simulink model "Test_Estimation_Effects"  (R2026a)
settings: Solver=FixedStepAuto  StopTime=SIM.StopTime  FixedStep=SIM.FixedStepSize
undefined symbols (not defined in the file): AP, AP_SRC, CMD, DES, DiscIntNeverNeededParam, drawAircraft, EST, F, Light, LIM, MAV, MIL, plotter, SIM, TRIM, WIND
libraries: simulink x11, matrix_library x2, aerolibwind2 x1
(part 1 of 2)
settings Model: Creator=emrec  LastModifiedBy=emrec

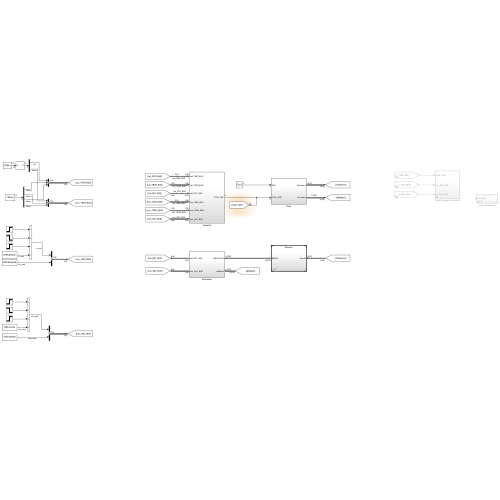
[thumbnail: Simulink's stored preview of the top-level diagram]
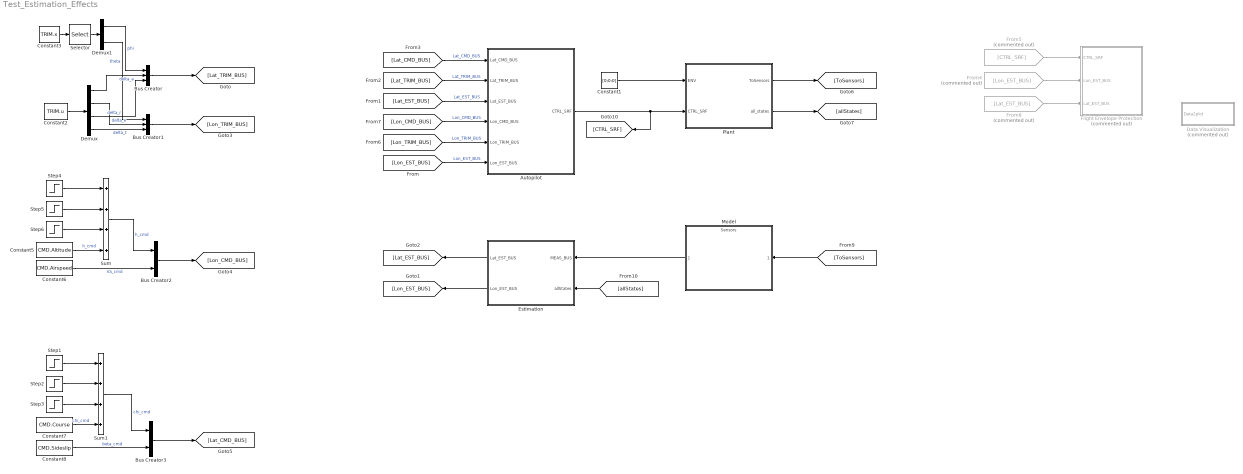
== system Test_Estimation_Effects ==
  Autopilot : Subsystem
  Bus Creator : BusCreator  Inputs=3
  Bus Creator1 : BusCreator  Inputs=3
  Bus Creator2 : BusCreator  Inputs=2
  Bus Creator3 : BusCreator  Inputs=2
  Constant1 : Constant  Value=[0;0;0]
  Constant2 : Constant  Value=TRIM.u
  Constant3 : Constant  Value=TRIM.x
  Constant5 : Constant  Value=CMD.Altitude
  Constant6 : Constant  Value=CMD.Airspeed
  Constant7 : Constant  Value=CMD.Course
  Constant8 : Constant  Value=CMD.Sideslip
  Data Visualization : Subsystem  Commented=on  Variant=on
  Demux : Demux
  Demux1 : Demux  Outputs=2
  Estimation : Subsystem  SystemSampleTime=EST.SamplingTime
  Flight Envelope Protection : Subsystem  Commented=on
  From4 : From  Commented=on  GotoTag=Lon_EST_BUS
  From5 : From  Commented=on  GotoTag=CTRL_SRF
  From8 : From  Commented=on  GotoTag=Lat_EST_BUS
  Model : ModelReference  ModelNameDialog=Sensors.slx  SimulationMode=Normal  ModelReferenceVersion=1.11
  Plant : Subsystem
  Selector : Selector  InputPortWidth=12  IndexOptions=Index vector (dialog)  Indices=[7,8]  OutputSizes=1
  Step1 : Step  Time=5  FinalValue=pi * 0.75  SampleTime=0
  Step2 : Step  Time=30  FinalValue=-pi * 0.75 * 2  SampleTime=0
  Step3 : Step  Time=75  FinalValue=pi * 0.75  SampleTime=0
  Step4 : Step  Time=10  FinalValue=10  SampleTime=0
  Step5 : Step  Time=50  FinalValue=-20  SampleTime=0
  Step6 : Step  Time=80  FinalValue=10  SampleTime=0
  Sum : Sum  Inputs=++++
  Sum1 : Sum  Inputs=++++
  wires:
  Constant1/1 -> Plant/1(ENV)
  Constant2/1 -> Demux/1
  Demux/1 -> Bus Creator/2  "delta_a"
  Demux/2 -> Bus Creator1/2  "delta_e"
  Demux/3 -> Bus Creator/3  "delta_r"
  Demux/4 -> Bus Creator1/3  "delta_t"
  Bus Creator/1 -> [Lat_TRIM_BUS]
  Bus Creator1/1 -> [Lon_TRIM_BUS]
  Constant3/1 -> Selector/1
  Selector/1 -> Demux1/1
  Demux1/1 -> Bus Creator/1  "phi"
  Demux1/2 -> Bus Creator1/1  "theta"
  Autopilot/1(CTRL_SRF) -> [CTRL_SRF], Plant/2(CTRL_SRF)
  [Lat_CMD_BUS] -> Autopilot/1(Lat_CMD_BUS)  "Lat_CMD_BUS"
  [Lat_TRIM_BUS] -> Autopilot/2(Lat_TRIM_BUS)  "Lat_TRIM_BUS"
  [Lat_EST_BUS] -> Autopilot/3(Lat_EST_BUS)  "Lat_EST_BUS"
  [Lon_CMD_BUS] -> Autopilot/4(Lon_CMD_BUS)  "Lon_CMD_BUS"
  [Lon_TRIM_BUS] -> Autopilot/5(Lon_TRIM_BUS)  "Lon_TRIM_BUS"
  [Lon_EST_BUS] -> Autopilot/6(Lon_EST_BUS)  "Lon_EST_BUS"
  From5/1 -> Flight Envelope Protection/1(CTRL_SRF)
  From4/1 -> Flight Envelope Protection/2(Lon_EST_BUS)
  From8/1 -> Flight Envelope Protection/3(Lat_EST_BUS)
  Model/1 -> Estimation/1(MEAS_BUS)
  Estimation/1(Lat_EST_BUS) -> [Lat_EST_BUS]
  Estimation/2(Lon_EST_BUS) -> [Lon_EST_BUS]
  Plant/1(ToSensors) -> [ToSensors]
  [ToSensors] -> Model/1
  Plant/2(all_states) -> [allStates]
  [allStates] -> Estimation/2(allStates)
  Bus Creator2/1 -> [Lon_CMD_BUS]
  Bus Creator3/1 -> [Lat_CMD_BUS]
  Sum/1 -> Bus Creator2/1  "h_cmd"
  Sum1/1 -> Bus Creator3/1  "chi_cmd"
  Constant6/1 -> Bus Creator2/2  "Va_cmd"
  Step6/1 -> Sum/3
  Constant5/1 -> Sum/4  "h_cmd"
  Step4/1 -> Sum/1
  Step1/1 -> Sum1/1
  Step2/1 -> Sum1/2
  Step5/1 -> Sum/2
  Constant7/1 -> Sum1/4  "chi_cmd"
  Step3/1 -> Sum1/3
  Constant8/1 -> Bus Creator3/2  "beta_cmd"

== system Test_Estimation_Effects/Autopilot ==
  Lat_CMD_BUS : Inport
  Lat_TRIM_BUS : Inport  Port=2
  Lat_EST_BUS : Inport  Port=3
  Lon_CMD_BUS : Inport  Port=4
  Lon_TRIM_BUS : Inport  Port=5
  Lon_EST_BUS : Inport  Port=6
  Lateral Autopilot : Subsystem
  Longitudinal Autopilot : Subsystem
  Mux1 : Mux
  CTRL_SRF : Outport
  wires:
  [delta_a] -> Mux1/1
  Lateral Autopilot/2(delta_r) -> [delta_r]
  [delta_t] -> Mux1/4
  Mux1/1 -> CTRL_SRF/1  "CTRL_SRF"
  Longitudinal Autopilot/1(delta_e) -> [delta_e]
  Longitudinal Autopilot/2(delta_t) -> [delta_t]
  [delta_e] -> Mux1/2
  Lon_CMD_BUS/1 -> Longitudinal Autopilot/1(Lon_CMD_BUS)
  [delta_r] -> Mux1/3
  Lateral Autopilot/1(delta_a) -> [delta_a]
  Lat_EST_BUS/1 -> Lateral Autopilot/3(Lat_EST_BUS)
  Lon_EST_BUS/1 -> Longitudinal Autopilot/3(Lon_EST_BUS)
  Lat_CMD_BUS/1 -> Lateral Autopilot/1(Lat_CMD_BUS)
  Lon_TRIM_BUS/1 -> Longitudinal Autopilot/2(Lon_TRIM_BUS)
  Lat_TRIM_BUS/1 -> Lateral Autopilot/2(Lat_TRIM_BUS)

== system Test_Estimation_Effects/Data Visualization ==
  note: 1) Add Subsystem or Model blocks as valid variant choices.
      | 2) You cannot connect blocks at this level. At simulation, connectivity is automatically
      | determined, based on the active variant and port name matching.
  Data2plot : Inport
  Data Storing : Subsystem  VariantControl=PLOTTING_MODEL == 2
  Online Plotting : Subsystem  VariantControl=PLOTTING_MODEL == 1

== system Test_Estimation_Effects/Estimation ==
  MEAS_BUS : Inport  OutDataTypeStr=Bus: SensorsMeasBus
  allStates : Inport  Port=2
  Model : ModelReference  ModelNameDialog=Estimation.slx  SimulationMode=Normal  ModelReferenceVersion=1.19
  Source Selection : Subsystem
  Unit Delay : UnitDelay  InitialCondition=EST.attitude_ekf.init_states  SampleTime=EST.SamplingTime
  Lat_EST_BUS : Outport
  Lon_EST_BUS : Outport  Port=2
  wires:
  MEAS_BUS/1 -> Model/1
  Model/1 -> Unit Delay/1  "attitude_ekf"
  Unit Delay/1 -> [EST_RES]
  Source Selection/1(Lat_EST_BUS) -> Lat_EST_BUS/1
  Source Selection/2(Lon_EST_BUS) -> Lon_EST_BUS/1
  [EST_RES] -> Source Selection/1(EST_RES)
  allStates/1 -> Source Selection/2(allStates)

== system Test_Estimation_Effects/Flight Envelope Protection ==
  CTRL_SRF : Inport
  Lon_EST_BUS : Inport  Port=2
  Lat_EST_BUS : Inport  Port=3
  Abs : Abs  SaturateOnIntegerOverflow=off
  Bus Selector : BusSelector  OutputSignals=p_nh_hat,Va_hat,theta_hat
  Compare To Constant : simulink/Logic and Bit Operations/Compare To Constant  relop=<  const=LIM.Altitude.min  OutDataTypeStr=boolean
  Compare To Constant1 : simulink/Logic and Bit Operations/Compare To Constant  relop=>  const=LIM.Altitude.max  OutDataTypeStr=boolean
  Compare To Constant2 : simulink/Logic and Bit Operations/Compare To Constant  relop=>  const=LIM.Airspeed.max  OutDataTypeStr=boolean
  Compare To Constant3 : simulink/Logic and Bit Operations/Compare To Constant  relop=>  const=LIM.Pitch.max  OutDataTypeStr=boolean
  Logical Operator : Logic  Operator=OR  Inputs=4  AllPortsSameDT=off  OutDataTypeStr=boolean
  Selector : Selector  InputPortWidth=2  IndexOptions=Index vector (dialog)  Indices=[2]  OutputSizes=1
  Stop Simulation : Stop
  wires:
  Lon_EST_BUS/1 -> Bus Selector/1
  Bus Selector/1 -> Selector/1  "<p_nh_hat>"
  Selector/1 -> Compare To Constant/1, Compare To Constant1/1
  Compare To Constant/1 -> Logical Operator/1  "crash"
  Compare To Constant1/1 -> Logical Operator/2  "excess_h"
  Compare To Constant2/1 -> Logical Operator/3  "excess_Va"
  Bus Selector/3 -> Abs/1  "<theta_hat>"
  Abs/1 -> Compare To Constant3/1
  Bus Selector/2 -> Compare To Constant2/1  "<Va_hat>"
  Compare To Constant3/1 -> Logical Operator/4  "excess_theta"
  Logical Operator/1 -> Stop Simulation/1

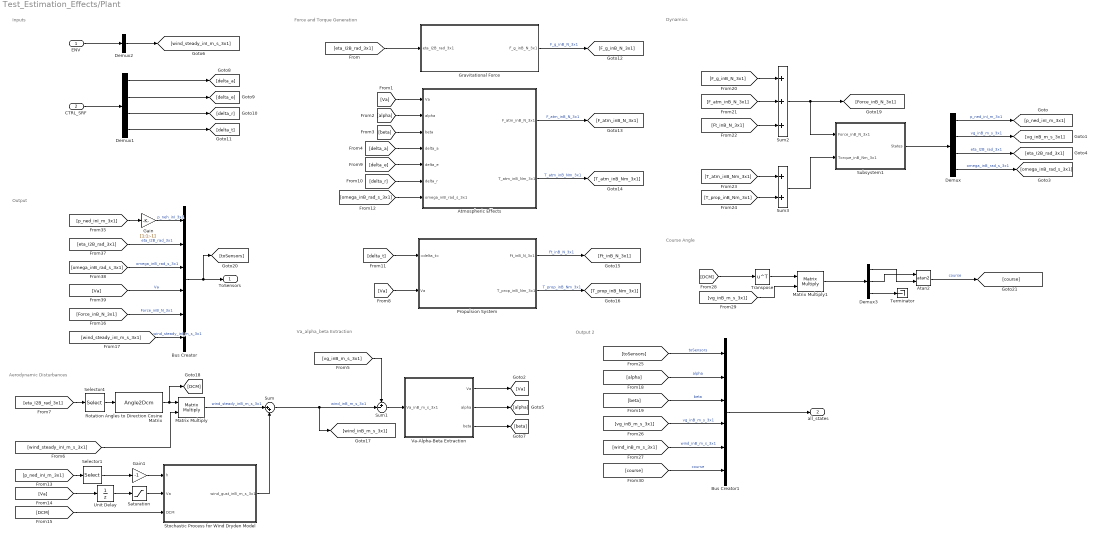
== system Test_Estimation_Effects/Plant ==
  note: Output 2
  note: Course Angle
  note: Aerodynamic Disturbances
  note: Force and Torque Generation
  note: Inputs
  note: Dynamics
  note: Va_alpha_beta Extraction
  note: Output
  ENV : Inport
  CTRL_SRF : Inport  Port=2
  Atan2 : Trigonometry  Operator=atan2
  Atmospheric Effects : Subsystem
  Bus Creator1 : BusCreator  Inputs=6
  Bus Creator : BusCreator  Inputs=6  OutDataTypeStr=Bus: SensorsInputsBus
  Demux : Demux
  Demux1 : Demux
  Demux2 : Demux  Outputs=1
  Demux3 : Demux  Outputs=3
  Gain : Gain  Gain=[1;1;-1]
  Gain1 : Gain  Gain=-1
  Gravitational Force : Subsystem
  Matrix Multiply : Product  Multiplication=Matrix(*)
  Matrix Multiply1 : Product  Multiplication=Matrix(*)
  Propulsion System : Subsystem
  Rotation Angles to Direction Cosine Matrix : Angle2Dcm
      settings: AttributesFormatString=Rotation Order: %<rotationOrder>
  Saturation : Saturate  UpperLimit=Inf  LowerLimit=0.1
  Selector1 : Selector  InputPortWidth=3  IndexOptions=Index vector (dialog)  Indices=3  OutputSizes=1
  Selector4 : Selector  InputPortWidth=3  IndexOptions=Index vector (dialog)  Indices=[3 2 1]  OutputSizes=1
  Stochastic Process for Wind Dryden Model : Subsystem
  Subsystem1 : Subsystem  mask{init_states=MAV.init_states, J_B_B=MAV.J_B_B, m=MAV.m}
      mask prompts: init_states "Initial state values"; J_B_B "Inertia matrix (Kg.m3)"; m "Mass (Kg)"
  Sum : Sum  Inputs=|++
  Sum1 : Sum  Inputs=+-|
  Sum2 : Sum  Inputs=+++
  Sum3 : Sum
  Terminator : Terminator
  Transpose : Math  Operator=transpose
  Unit Delay : UnitDelay  SampleTime=-1
  Va-Alpha-Beta Extraction : Subsystem
  ToSensors : Outport
  all_states : Outport  Port=2
  wires:
  Bus Creator/1 -> [toSensors], ToSensors/1
  [omega_inB_rad_s_3x1] -> Bus Creator/3  "omega_inB_rad_s_3x1"
  [eta_I2B_rad_3x1] -> Bus Creator/2  "eta_I2B_rad_3x1"
  [p_ned_inI_m_3x1] -> Gain/1
  [Va] -> Propulsion System/2(Va)
  [delta_t] -> Propulsion System/1(<delta_t>)
  Propulsion System/1(Ft_inB_N_3x1) -> [Ft_inB_N_3x1]  "Ft_inB_N_3x1"
  Propulsion System/2(T_prop_inB_Nm_3x1) -> [T_prop_inB_Nm_3x1]  "T_prop_inB_Nm_3x1"
  [T_prop_inB_Nm_3x1] -> Sum3/2
  [T_atm_inB_Nm_3x1] -> Sum3/1
  [Ft_inB_N_3x1] -> Sum2/3
  [F_atm_inB_N_3x1] -> Sum2/2
  [F_g_inB_N_3x1] -> Sum2/1
  Gravitational Force/1(F_g_inB_N_3x1) -> [F_g_inB_N_3x1]  "F_g_inB_N_3x1"
  Atmospheric Effects/1(F_atm_inB_N_3x1) -> [F_atm_inB_N_3x1]  "F_atm_inB_N_3x1"
  Atmospheric Effects/2(T_atm_inB_Nm_3x1) -> [T_atm_inB_Nm_3x1]  "T_atm_inB_Nm_3x1"
  Demux1/2 -> [delta_e]
  ENV/1 -> Demux2/1
  Sum1/1 -> Va-Alpha-Beta Extraction/1(Va_inB_m_s_3x1)
  [wind_steady_inI_m_s_3x1] -> Matrix Multiply/2
  Demux2/1 -> [wind_steady_inI_m_s_3x1]
  Selector4/1 -> Rotation Angles to Direction Cosine Matrix/1
  Demux1/4 -> [delta_t]
  [Va] -> Atmospheric Effects/1(Va)
  Va-Alpha-Beta Extraction/1(Va) -> [Va]
  Demux/4 -> [omega_inB_rad_s_3x1]  "omega_inB_rad_s_3x1"
  [delta_r] -> Atmospheric Effects/6(delta_r)
  [delta_a] -> Atmospheric Effects/4(delta_a)
  Matrix Multiply/1 -> Sum/1  "wind_steady_inB_m_s_3x1"
  [delta_e] -> Atmospheric Effects/5(delta_e)
  Subsystem1/1(States) -> Demux/1
  Va-Alpha-Beta Extraction/3(beta) -> [beta]
  Demux/1 -> [p_ned_inI_m_3x1]  "p_ned_inI_m_3x1"
  CTRL_SRF/1 -> Demux1/1
  Demux1/1 -> [delta_a]
  Demux/3 -> [eta_I2B_rad_3x1]  "eta_I2B_rad_3x1"
  Sum/1 -> Sum1/2, [wind_inB_m_s_3x1]  "wind_inB_m_s_3x1"
  [vg_inB_m_s_3x1] -> Sum1/1
  Demux/2 -> [vg_inB_m_s_3x1]  "vg_inB_m_s_3x1"
  [eta_I2B_rad_3x1] -> Selector4/1
  Rotation Angles to Direction Cosine Matrix/1 -> [DCM], Matrix Multiply/1
  [eta_I2B_rad_3x1] -> Gravitational Force/1(eta_I2B_rad_3x1)
  Sum3/1 -> Subsystem1/2(Torque_inB_Nm_3x1)
  Va-Alpha-Beta Extraction/2(alpha) -> [alpha]
  Sum2/1 -> Subsystem1/1(Force_inB_N_3x1), [Force_inB_N_3x1]
  [alpha] -> Atmospheric Effects/2(alpha)
  [beta] -> Atmospheric Effects/3(beta)
  Demux1/3 -> [delta_r]
  [omega_inB_rad_s_3x1] -> Atmospheric Effects/7(omega_inB_rad_s_3x1)
  [Va] -> Bus Creator/4  "Va"
  Gain/1 -> Bus Creator/1  "p_neh_inI_3x1"
  [p_ned_inI_m_3x1] -> Selector1/1
  [Va] -> Unit Delay/1
  [DCM] -> Stochastic Process for Wind Dryden Model/3(DCM)
  Selector1/1 -> Gain1/1
  Gain1/1 -> Stochastic Process for Wind Dryden Model/1(h)
  Unit Delay/1 -> Saturation/1
  Saturation/1 -> Stochastic Process for Wind Dryden Model/2(Va)
  [Force_inB_N_3x1] -> Bus Creator/5  "Force_inB_N_3x1"
  [wind_steady_inI_m_s_3x1] -> Bus Creator/6  "wind_steady_inI_m_s_3x1"
  [toSensors] -> Bus Creator1/1  "toSensors"
  [alpha] -> Bus Creator1/2  "alpha"
  [beta] -> Bus Creator1/3  "beta"
  [vg_inB_m_s_3x1] -> Bus Creator1/4  "vg_inB_m_s_3x1"
  [wind_inB_m_s_3x1] -> Bus Creator1/5  "wind_inB_m_s_3x1"
  Bus Creator1/1 -> all_states/1
  Stochastic Process for Wind Dryden Model/1(wind_gust_inB_m_s_3x1) -> Sum/2
  Demux3/3 -> Terminator/1
  [vg_inB_m_s_3x1] -> Matrix Multiply1/2
  Demux3/1 -> Atan2/2
  Matrix Multiply1/1 -> Demux3/1
  Atan2/1 -> [course]  "course"
  Transpose/1 -> Matrix Multiply1/1
  Demux3/2 -> Atan2/1
  [DCM] -> Transpose/1
  [course] -> Bus Creator1/6  "course"

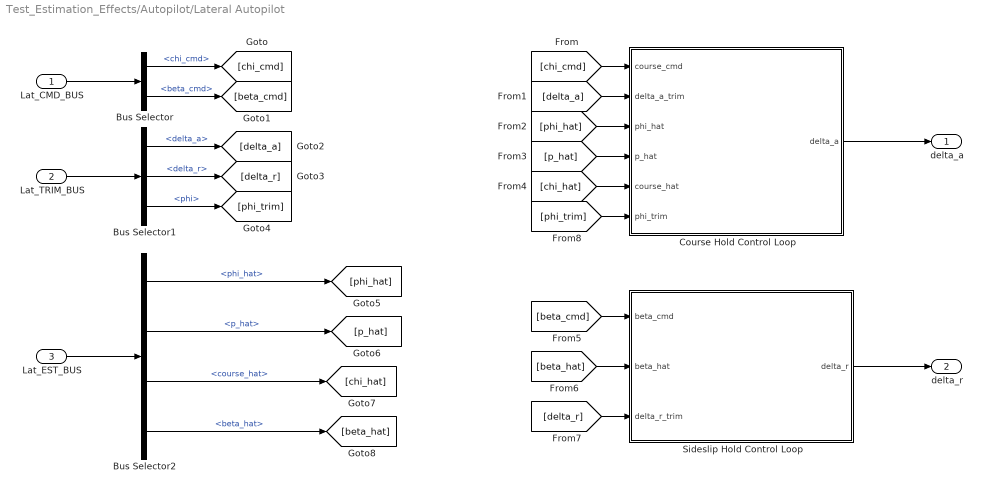
== system Test_Estimation_Effects/Autopilot/Lateral Autopilot ==
  Lat_CMD_BUS : Inport
  Lat_TRIM_BUS : Inport  Port=2
  Lat_EST_BUS : Inport  Port=3
  Bus Selector : BusSelector  OutputSignals=chi_cmd,beta_cmd
  Bus Selector1 : BusSelector  OutputSignals=delta_a,delta_r,phi
  Bus Selector2 : BusSelector  OutputSignals=phi_hat,p_hat,course_hat,beta_hat
  Course Hold Control Loop : Subsystem
  Sideslip Hold Control Loop : Subsystem
  delta_a : Outport
  delta_r : Outport  Port=2
  wires:
  Sideslip Hold Control Loop/1(delta_r) -> delta_r/1
  Course Hold Control Loop/1(delta_a) -> delta_a/1
  Lat_CMD_BUS/1 -> Bus Selector/1
  Bus Selector/1 -> [chi_cmd]  "<chi_cmd>"
  Bus Selector/2 -> [beta_cmd]  "<beta_cmd>"
  Lat_TRIM_BUS/1 -> Bus Selector1/1
  Bus Selector1/1 -> [delta_a]  "<delta_a>"
  Bus Selector1/2 -> [delta_r]  "<delta_r>"
  Lat_EST_BUS/1 -> Bus Selector2/1
  Bus Selector2/2 -> [p_hat]  "<p_hat>"
  Bus Selector2/3 -> [chi_hat]  "<course_hat>"
  Bus Selector2/4 -> [beta_hat]  "<beta_hat>"
  [chi_cmd] -> Course Hold Control Loop/1(course_cmd)
  [delta_a] -> Course Hold Control Loop/2(delta_a_trim)
  [phi_hat] -> Course Hold Control Loop/3(phi_hat)
  [p_hat] -> Course Hold Control Loop/4(p_hat)
  [chi_hat] -> Course Hold Control Loop/5(course_hat)
  [beta_cmd] -> Sideslip Hold Control Loop/1(beta_cmd)
  [beta_hat] -> Sideslip Hold Control Loop/2(beta_hat)
  [delta_r] -> Sideslip Hold Control Loop/3(delta_r_trim)
  Bus Selector1/3 -> [phi_trim]  "<phi>"
  [phi_trim] -> Course Hold Control Loop/6(phi_trim)
  Bus Selector2/1 -> [phi_hat]  "<phi_hat>"

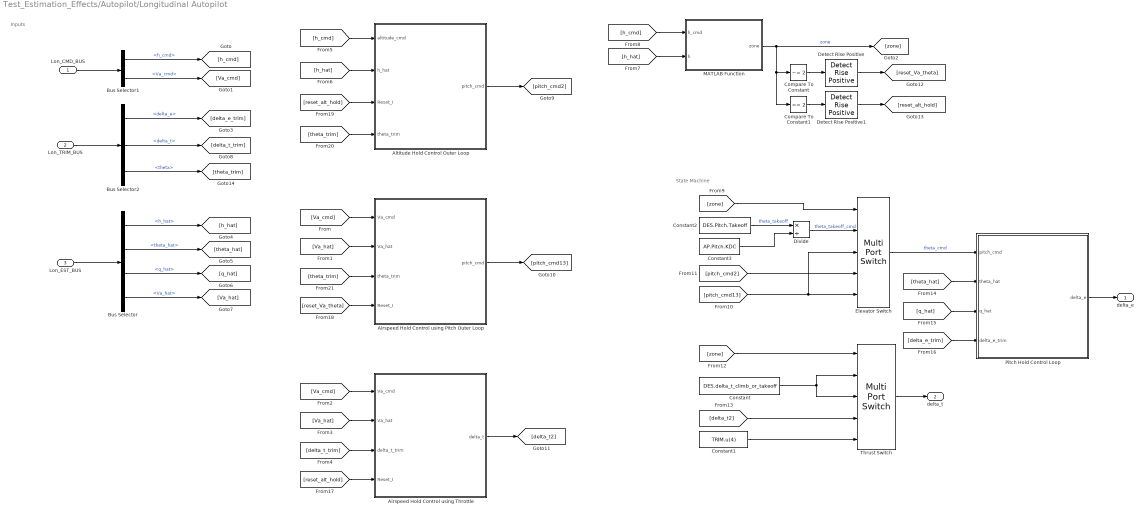
== system Test_Estimation_Effects/Autopilot/Longitudinal Autopilot ==
  note: Inputs
  note: State Machine
  Lon_CMD_BUS : Inport
  Lon_TRIM_BUS : Inport  Port=2
  Lon_EST_BUS : Inport  Port=3
  Airspeed Hold Control using Pitch Outer Loop : Subsystem
  "Airspeed Hold Control using Throttle " : Subsystem
  Altitude Hold Control Outer Loop : Subsystem
  Bus Selector : BusSelector  OutputSignals=h_hat,theta_hat,q_hat,Va_hat
  Bus Selector1 : BusSelector  OutputSignals=h_cmd,Va_cmd
  Bus Selector2 : BusSelector  OutputSignals=delta_e,delta_t,theta
  Compare To Constant : simulink/Logic and Bit Operations/Compare To Constant  relop=~=  const=2  OutDataTypeStr=boolean
  Compare To Constant1 : simulink/Logic and Bit Operations/Compare To Constant  relop===  const=2  OutDataTypeStr=boolean
  Constant : Constant  Value=DES.delta_t_climb_or_takeoff
  Constant1 : Constant  Value=TRIM.u(4)
  Constant2 : Constant  Value=DES.Pitch.Takeoff
  Constant3 : Constant  Value=AP.Pitch.KDC
  Detect Rise Positive : simulink/Logic and Bit Operations/Detect Rise Positive  vinit=0  OutDataTypeStr=boolean
  Detect Rise Positive1 : simulink/Logic and Bit Operations/Detect Rise Positive  vinit=0  OutDataTypeStr=boolean
  Divide : Product  Inputs=*/
  Elevator Switch : MultiPortSwitch  DataPortOrder=Zero-based contiguous  Inputs=4  zeroidx=on  SaturateOnIntegerOverflow=off  InputSameDT=off
  MATLAB Function : MATLAB Function  TreatAsAtomicUnit=on  SystemSampleTime=SIM.FixedStepSize
  Pitch Hold Control Loop : Subsystem
  Thrust Switch : MultiPortSwitch  DataPortOrder=Zero-based contiguous  Inputs=4  zeroidx=on  SaturateOnIntegerOverflow=off  InputSameDT=off
  delta_e : Outport
  delta_t : Outport  Port=2
  wires:
  Pitch Hold Control Loop/1(delta_e) -> delta_e/1
  [h_hat] -> MATLAB Function/2(h)
  Constant/1 -> Thrust Switch/2, Thrust Switch/3
  Constant1/1 -> Thrust Switch/5
  Thrust Switch/1 -> delta_t/1
  Constant2/1 -> Divide/1  "theta_takeoff"
  Constant3/1 -> Divide/2
  Divide/1 -> Elevator Switch/2  "theta_takeoff_cmd"
  [Va_cmd] -> Airspeed Hold Control using Pitch Outer Loop/1(Va_cmd)
  [Va_hat] -> Airspeed Hold Control using Pitch Outer Loop/2(Va_hat)
  Lon_EST_BUS/1 -> Bus Selector/1
  Bus Selector/1 -> [h_hat]  "<h_hat>"
  Bus Selector/2 -> [theta_hat]  "<theta_hat>"
  Bus Selector/3 -> [q_hat]  "<q_hat>"
  Bus Selector/4 -> [Va_hat]  "<Va_hat>"
  Lon_CMD_BUS/1 -> Bus Selector1/1
  Bus Selector1/1 -> [h_cmd]  "<h_cmd>"
  Bus Selector1/2 -> [Va_cmd]  "<Va_cmd>"
  Bus Selector2/1 -> [delta_e_trim]  "<delta_e>"
  Lon_TRIM_BUS/1 -> Bus Selector2/1
  Bus Selector2/2 -> [delta_t_trim]  "<delta_t>"
  [Va_cmd] -> "Airspeed Hold Control using Throttle "/1(Va_cmd)
  [Va_hat] -> "Airspeed Hold Control using Throttle "/2(Va_hat)
  [delta_t_trim] -> "Airspeed Hold Control using Throttle "/3(delta_t_trim)
  [h_cmd] -> Altitude Hold Control Outer Loop/1(altitude_cmd)
  [h_hat] -> Altitude Hold Control Outer Loop/2(h_hat)
  Altitude Hold Control Outer Loop/1(pitch_cmd) -> [pitch_cmd2]
  Airspeed Hold Control using Pitch Outer Loop/1(pitch_cmd) -> [pitch_cmd13]
  "Airspeed Hold Control using Throttle "/1(delta_t) -> [delta_t2]
  [h_cmd] -> MATLAB Function/1(h_cmd)
  [zone] -> Elevator Switch/1
  [pitch_cmd13] -> Elevator Switch/5, Elevator Switch/3
  [pitch_cmd2] -> Elevator Switch/4
  [zone] -> Thrust Switch/1
  [delta_t2] -> Thrust Switch/4
  [theta_hat] -> Pitch Hold Control Loop/2(theta_hat)
  [q_hat] -> Pitch Hold Control Loop/3(q_hat)
  [delta_e_trim] -> Pitch Hold Control Loop/4(delta_e_trim)
  Compare To Constant/1 -> Detect Rise Positive/1
  Compare To Constant1/1 -> Detect Rise Positive1/1
  Detect Rise Positive/1 -> [reset_Va_theta]
  Detect Rise Positive1/1 -> [reset_alt_hold]
  [reset_alt_hold] -> "Airspeed Hold Control using Throttle "/4(Reset_I)
  [reset_Va_theta] -> Airspeed Hold Control using Pitch Outer Loop/4(Reset_I)
  [reset_alt_hold] -> Altitude Hold Control Outer Loop/3(Reset_I)
  Bus Selector2/3 -> [theta_trim]  "<theta>"
  [theta_trim] -> Altitude Hold Control Outer Loop/4(theta_trim)
  [theta_trim] -> Airspeed Hold Control using Pitch Outer Loop/3(theta_trim)
  MATLAB Function/1(zone) -> [zone], Compare To Constant1/1, Compare To Constant/1  "zone"
  Elevator Switch/1 -> Pitch Hold Control Loop/1(pitch_cmd)  "theta_cmd"

== system Test_Estimation_Effects/Data Visualization/Data Storing ==
  Data2plot : Inport
  To Workspace : ToWorkspace  VariableName=simout  SampleTime=-1
  wires:
  Data2plot/1 -> To Workspace/1

== system Test_Estimation_Effects/Data Visualization/Online Plotting ==
  Data2plot : Inport
  Aircraft Body Animation : MATLABFcn  MATLABFcn=drawAircraft(u)  OutputDimensions=0
  Clock : Clock
  Mux : Mux  Inputs=2
  Plot Graphs : MATLABFcn  MATLABFcn=plotter(u)  OutputDimensions=0
  Selector : Selector  InputPortWidth=38  IndexOptions=Index vector (dialog)  Indices=[1:12]  OutputSizes=1
  wires:
  Mux/1 -> Aircraft Body Animation/1
  Clock/1 -> Mux/2
  Selector/1 -> Mux/1
  Data2plot/1 -> Plot Graphs/1, Selector/1

== system Test_Estimation_Effects/Estimation/Source Selection ==
  EST_RES : Inport
  allStates : Inport  Port=2
  Plant Signals Adapter : Subsystem
  Source Selector : Subsystem
  Lat_EST_BUS : Outport
  Lon_EST_BUS : Outport  Port=2
  wires:
  allStates/1 -> Plant Signals Adapter/1(allStates)
  EST_RES/1 -> Source Selector/1(EST_RES)
  Plant Signals Adapter/2(GPS_PLANT_BUS) -> Source Selector/3(GPS_PLANT_BUS)
  Plant Signals Adapter/3(Press_Ang_Vel_RES_PLANT_BUS) -> Source Selector/4(Press_Ang_Vel_RES_PLANT_BUS)
  Source Selector/2(Lon_EST_BUS) -> Lon_EST_BUS/1  "Lon_EST_BUS"
  Source Selector/1(Lat_EST_BUS) -> Lat_EST_BUS/1  "Lat_EST_BUS"
  Plant Signals Adapter/1(Attitude_PLANT_VEC) -> Source Selector/2(Attitude_PLANT_VEC)
  Plant Signals Adapter/4(OTHER_PLANT_BUS) -> Source Selector/5(OTHER_PLANT_BUS)

== system Test_Estimation_Effects/Plant/Atmospheric Effects ==
  Va : Inport
  alpha : Inport  Port=2
  beta : Inport  Port=3
  delta_a : Inport  Port=4
  delta_e : Inport  Port=5
  delta_r : Inport  Port=6
  omega_inB_rad_s_3x1 : Inport  Port=7
  Aerodynamic Effect on Latitude Motion : Subsystem
  Aerodynamic Effect on Longitudinal Motion : Subsystem
  Mux1 : Mux  Inputs=2
  Selector : Selector  InputPortWidth=3  IndexOptions=Index vector (dialog)  Indices=[2]  OutputSizes=1
  Selector1 : Selector  InputPortWidth=3  IndexOptions=Index vector (dialog)  Indices=[1 3]  OutputSizes=1
  Selector2 : Selector  InputPortWidth=6  IndexOptions=Index vector (dialog)  Indices=[1 4 2]  OutputSizes=1
  Selector3 : Selector  InputPortWidth=6  IndexOptions=Index vector (dialog)  Indices=[5 3 6]  OutputSizes=1
  F_atm_inB_N_3x1 : Outport
  T_atm_inB_Nm_3x1 : Outport  Port=2
  wires:
  Mux1/1 -> Selector3/1, Selector2/1
  Selector2/1 -> F_atm_inB_N_3x1/1  "F_atm_inB_N_3x1"
  delta_e/1 -> Aerodynamic Effect on Longitudinal Motion/1(delta_e)
  delta_a/1 -> Aerodynamic Effect on Latitude Motion/1(delta_a)
  Aerodynamic Effect on Longitudinal Motion/1(Fx_Fz_Tq_inB) -> Mux1/1
  alpha/1 -> Aerodynamic Effect on Longitudinal Motion/3(alpha)
  Aerodynamic Effect on Latitude Motion/1(Fy_Tp_Tr_inB) -> Mux1/2
  delta_r/1 -> Aerodynamic Effect on Latitude Motion/2(delta_r)
  omega_inB_rad_s_3x1/1 -> Selector1/1, Selector/1
  Va/1 -> Aerodynamic Effect on Latitude Motion/5(Va), Aerodynamic Effect on Longitudinal Motion/4(Va)
  beta/1 -> Aerodynamic Effect on Latitude Motion/3(beta)
  Selector3/1 -> T_atm_inB_Nm_3x1/1  "T_atm_inB_Nm_3x1"
  Selector/1 -> Aerodynamic Effect on Longitudinal Motion/2(q)
  Selector1/1 -> Aerodynamic Effect on Latitude Motion/4(p_r)

== system Test_Estimation_Effects/Plant/Gravitational Force ==
  eta_I2B_rad_3x1 : Inport
  Constant : Constant  Value=MAV.m * MAV.g
  Product : Product
  R_B_I_c3 : MATLAB Function  TreatAsAtomicUnit=on
  F_g_inB_N_3x1 : Outport
  wires:
  eta_I2B_rad_3x1/1 -> R_B_I_c3/1(u)
  R_B_I_c3/1(y) -> Product/1
  Constant/1 -> Product/2  "F_g_inI_N_3x1"
  Product/1 -> F_g_inB_N_3x1/1  "F_g_inB_N_3x1"

== system Test_Estimation_Effects/Plant/Propulsion System ==
  <delta_t> : Inport
  Va : Inport  Port=2
  Gain2 : Gain  Gain=MAV.K_motor
  Gain3 : Gain  Gain=MAV.S_prop * MAV.C_prop * MAV.rho/ 2
  Gain4 : Gain  Gain=-MAV.K_t_prop
  Gain5 : Gain  Gain=MAV.K_omega
  Square1 : Math  Operator=square
  Square2 : Math  Operator=square
  Square3 : Math  Operator=square
  Sum2 : Sum  Inputs=|+-
  vectorize_e1 : Gain  Gain=[1;0;0]
  vectorize_e2 : Gain  Gain=[1;0;0]
  Ft_inB_N_3x1 : Outport
  T_prop_inB_Nm_3x1 : Outport  Port=2
  wires:
  Gain5/1 -> Square3/1  "V_exit"
  Square3/1 -> Gain4/1
  vectorize_e2/1 -> T_prop_inB_Nm_3x1/1  "T_prop_inB_Nm_3x1"
  Va/1 -> Square2/1
  <delta_t>/1 -> Gain5/1, Gain2/1
  Gain3/1 -> Ft_inB_N_3x1/1  "Ft_inB_N_3x1"
  vectorize_e1/1 -> Gain3/1
  Square2/1 -> Sum2/2
  Sum2/1 -> vectorize_e1/1
  Gain4/1 -> vectorize_e2/1
  Square1/1 -> Sum2/1
  Gain2/1 -> Square1/1  "V_exit"

== system Test_Estimation_Effects/Plant/Stochastic Process for Wind Dryden Model ==
  h : Inport
  Va : Inport  Port=2
  DCM : Inport  Port=3
  Band-Limited White Noise : simulink/Sources/Band-Limited White Noise  Commented=on  Cov=[WIND.Dryden.Pu]  Ts=SIM.IntegratorSamplingTime  seed=[WIND.Dryden.seed_u]
  Band-Limited White Noise1 : simulink/Sources/Band-Limited White Noise  Commented=on  Cov=[WIND.Dryden.Pv]  Ts=SIM.FixedStepSize  seed=[WIND.Dryden.seed_v]
  Band-Limited White Noise2 : simulink/Sources/Band-Limited White Noise  Commented=on  Cov=[WIND.Dryden.Pw]  Ts=SIM.FixedStepSize  seed=[WIND.Dryden.seed_w]
  Dryden Wind Turbulence Model (Continuous (+q +r)) : aerolibwind2/Dryden Wind Turbulence Model  (Continuous (+q -r))  units=Metric (MKS)  spec=MIL-F-8785C  model=Continuous Dryden (+q +r)  W20=WIND.Dryden.Va_at6m  Wdeg=WIND.Dryden.dir_at6m_deg  TurbProb=10^-2 - Light  L_high=533.4  Wingspan=MAV.b  ts=SIM.FixedStepSize  Seed=[WIND.Dryden.seed_u, WIND.Dryden.seed_v, WIND.Dryden.seed_w, 5433]  T_on=on
      settings: LibrarySourceBlock=|
      | aerolibwind2/Dryden Wind Turbulence Model
      | (Continuous (+q +r))
  Hus : TransferFcn  Commented=on  Numerator=WIND.Dryden.Hus.Numerator{:}  Denominator=WIND.Dryden.Hus.Denominator{:}
  Hvs : TransferFcn  Commented=on  Numerator=WIND.Dryden.Hvs.Numerator{:}  Denominator=WIND.Dryden.Hvs.Denominator{:}
  Hws : TransferFcn  Commented=on  Numerator=WIND.Dryden.Hws.Numerator{:}  Denominator=WIND.Dryden.Hws.Denominator{:}
  Mux : Mux  Commented=on  Inputs=3
  Terminator : Terminator
  wind_gust_inB_m_s_3x1 : Outport
  wires:
  Band-Limited White Noise2/1 -> Hws/1
  Band-Limited White Noise/1 -> Hus/1
  Band-Limited White Noise1/1 -> Hvs/1
  Hus/1 -> Mux/1
  Hvs/1 -> Mux/2
  Hws/1 -> Mux/3
  h/1 -> Dryden Wind Turbulence Model (Continuous (+q +r))/1
  Va/1 -> Dryden Wind Turbulence Model (Continuous (+q +r))/2
  DCM/1 -> Dryden Wind Turbulence Model (Continuous (+q +r))/3
  Dryden Wind Turbulence Model (Continuous (+q +r))/1 -> wind_gust_inB_m_s_3x1/1
  Dryden Wind Turbulence Model (Continuous (+q +r))/2 -> Terminator/1

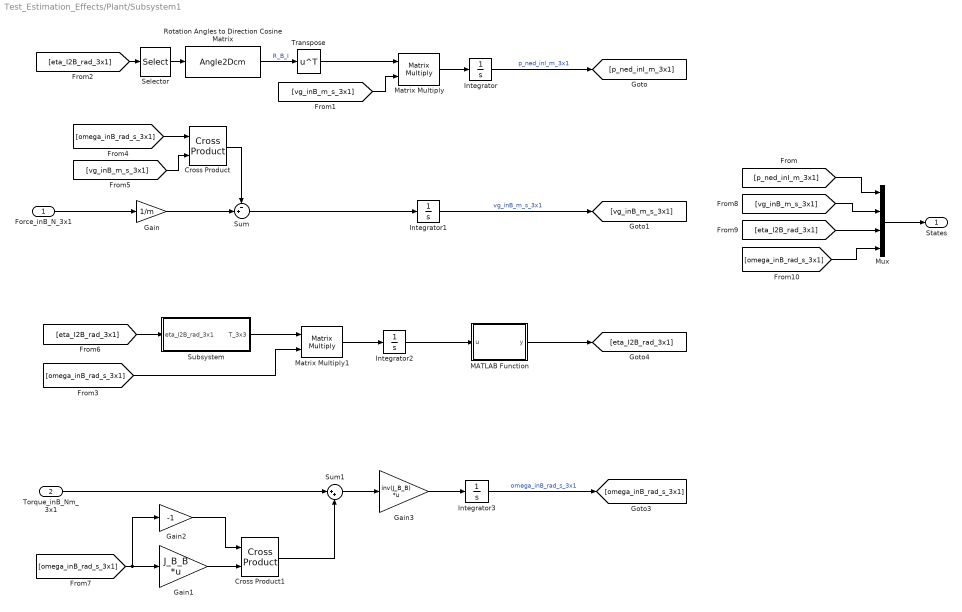
== system Test_Estimation_Effects/Plant/Subsystem1 ==
  Force_inB_N_3x1 : Inport
  Torque_inB_Nm_3x1 : Inport  Port=2
  Cross Product : matrix_library/Cross Product
  Cross Product1 : matrix_library/Cross Product
  Gain : Gain  Gain=1/m
  Gain1 : Gain  Gain=J_B_B  Multiplication=Matrix(K*u)
  Gain2 : Gain  Gain=-1
  Gain3 : Gain  Gain=inv(J_B_B)  Multiplication=Matrix(K*u)
  Integrator : Integrator  InitialCondition=init_states(1:3)
  Integrator1 : Integrator  InitialCondition=init_states(4:6)
  Integrator2 : Integrator  InitialCondition=init_states(7:9)
  Integrator3 : Integrator  InitialCondition=init_states(10:12)
  MATLAB Function : MATLAB Function  TreatAsAtomicUnit=on
  Matrix Multiply : Product  Multiplication=Matrix(*)
  Matrix Multiply1 : Product  Multiplication=Matrix(*)
  Mux : Mux
  Rotation Angles to Direction Cosine Matrix : Angle2Dcm
      settings: AttributesFormatString=Rotation Order: %<rotationOrder>
  Selector : Selector  InputPortWidth=3  IndexOptions=Index vector (dialog)  Indices=[3;2;1]  OutputSizes=1
  Subsystem : Subsystem
  Sum : Sum  Inputs=-+|
  Sum1 : Sum  Inputs=|++
  Transpose : Math  Operator=transpose
  States : Outport
  wires:
  MATLAB Function/1(y) -> [eta_I2B_rad_3x1]
  Gain3/1 -> Integrator3/1
  [p_ned_inI_m_3x1] -> Mux/1
  [omega_inB_rad_s_3x1] -> Cross Product/1
  Matrix Multiply1/1 -> Integrator2/1
  Gain1/1 -> Cross Product1/2
  [eta_I2B_rad_3x1] -> Subsystem/1(eta_I2B_rad_3x1)
  [omega_inB_rad_s_3x1] -> Matrix Multiply1/2
  Integrator1/1 -> [vg_inB_m_s_3x1]  "vg_inB_m_s_3x1"
  [vg_inB_m_s_3x1] -> Cross Product/2
  Selector/1 -> Rotation Angles to Direction Cosine Matrix/1
  [eta_I2B_rad_3x1] -> Selector/1
  Cross Product/1 -> Sum/1
  Integrator/1 -> [p_ned_inI_m_3x1]  "p_ned_inI_m_3x1"
  Matrix Multiply/1 -> Integrator/1
  Force_inB_N_3x1/1 -> Gain/1
  Rotation Angles to Direction Cosine Matrix/1 -> Transpose/1  "R_B_I"
  [omega_inB_rad_s_3x1] -> Gain2/1, Gain1/1
  Mux/1 -> States/1
  [omega_inB_rad_s_3x1] -> Mux/4
  Transpose/1 -> Matrix Multiply/1
  Integrator3/1 -> [omega_inB_rad_s_3x1]  "omega_inB_rad_s_3x1"
  [vg_inB_m_s_3x1] -> Matrix Multiply/2
  [eta_I2B_rad_3x1] -> Mux/3
  Torque_inB_Nm_3x1/1 -> Sum1/1
  Gain2/1 -> Cross Product1/1
  Sum1/1 -> Gain3/1
  Integrator2/1 -> MATLAB Function/1(u)
  [vg_inB_m_s_3x1] -> Mux/2
  Subsystem/1(T_3x3) -> Matrix Multiply1/1
  Cross Product1/1 -> Sum1/2
  Sum/1 -> Integrator1/1
  Gain/1 -> Sum/2

== system Test_Estimation_Effects/Plant/Va-Alpha-Beta Extraction ==
  note: To avoid zero division problem.
      | This logic and threshold is recommended by gemini.
  note: Va >= ||vr|| -> Va = 0 -> vr = 0
  Va_inB_m_s_3x1 : Inport
  Asin : Trigonometry  Operator=asin
  Constant : Constant
  Demux : Demux  Outputs=3
  Divide1 : Product  Inputs=*/
  Switch : Switch  Criteria=u2 > Threshold  SaturateOnIntegerOverflow=off  InputSameDT=off
  Trigonometric Function : Trigonometry  Operator=atan2  OutputSignalType=real
  norm2 : Subsystem
  Va : Outport
  alpha : Outport  Port=2
  beta : Outport  Port=3
  wires:
  Va_inB_m_s_3x1/1 -> norm2/1(Va_inB_m_s_3x1), Demux/1
  Demux/1 -> Trigonometric Function/2  "ur"
  Demux/2 -> Divide1/1  "vr"
  Demux/3 -> Trigonometric Function/1  "wr"
  norm2/1(Va) -> Switch/2, Switch/1, Va/1  "Va"
  Divide1/1 -> Asin/1
  Asin/1 -> beta/1
  Trigonometric Function/1 -> alpha/1
  Constant/1 -> Switch/3
  Switch/1 -> Divide1/2

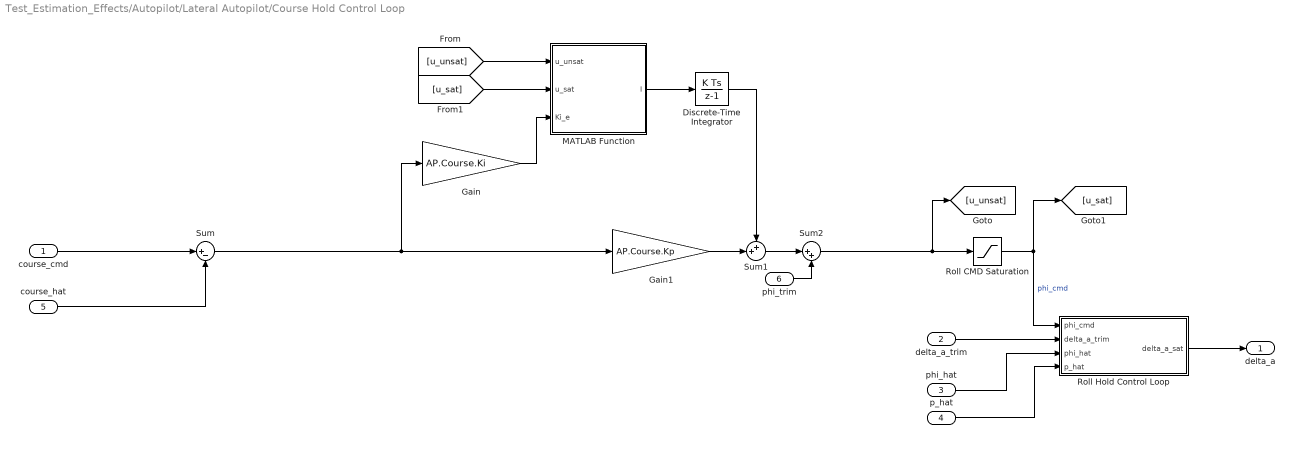
== system Test_Estimation_Effects/Autopilot/Lateral Autopilot/Course Hold Control Loop ==
  course_cmd : Inport
  delta_a_trim : Inport  Port=2
  phi_hat : Inport  Port=3
  p_hat : Inport  Port=4
  course_hat : Inport  Port=5
  phi_trim : Inport  Port=6
  Discrete-Time Integrator : DiscreteIntegrator  SampleTime=SIM.IntegratorSamplingTime  ICPrevOutput=DiscIntNeverNeededParam  ICPrevScaledInput=DiscIntNeverNeededParam
  Gain : Gain  Gain=AP.Course.Ki
  Gain1 : Gain  Gain=AP.Course.Kp
  MATLAB Function : MATLAB Function  TreatAsAtomicUnit=on
  "Roll CMD Saturation " : Saturate  UpperLimit=DES.Roll.max  LowerLimit=-DES.Roll.max
  Roll Hold Control Loop : Subsystem
  Sum : Sum  Inputs=|+-
  Sum1 : Sum  Inputs=++|
  Sum2 : Sum  Inputs=|++
  delta_a : Outport
  wires:
  p_hat/1 -> Roll Hold Control Loop/4(p_hat)
  Discrete-Time Integrator/1 -> Sum1/1
  Sum/1 -> Gain1/1, Gain/1
  Gain1/1 -> Sum1/2
  phi_hat/1 -> Roll Hold Control Loop/3(phi_hat)
  course_cmd/1 -> Sum/1
  course_hat/1 -> Sum/2
  delta_a_trim/1 -> Roll Hold Control Loop/2(delta_a_trim)
  Roll Hold Control Loop/1(delta_a_sat) -> delta_a/1
  Sum2/1 -> [u_unsat], "Roll CMD Saturation "/1
  "Roll CMD Saturation "/1 -> Roll Hold Control Loop/1(phi_cmd), [u_sat]  "phi_cmd"
  Gain/1 -> MATLAB Function/3(Ki_e)
  [u_unsat] -> MATLAB Function/1(u_unsat)
  [u_sat] -> MATLAB Function/2(u_sat)
  MATLAB Function/1(I) -> Discrete-Time Integrator/1
  Sum1/1 -> Sum2/1
  phi_trim/1 -> Sum2/2

== system Test_Estimation_Effects/Autopilot/Lateral Autopilot/Sideslip Hold Control Loop ==
  beta_cmd : Inport
  beta_hat : Inport  Port=2
  delta_r_trim : Inport  Port=3
  Gain : Gain  Gain=-AP.Sideslip.Ki
  Gain1 : Gain  Gain=-AP.Sideslip.Kp
  MATLAB Function : MATLAB Function  TreatAsAtomicUnit=on
  Rudder Saturation : Saturate  UpperLimit=DES.delta_r_max  LowerLimit=-DES.delta_r_max
  Sideslip I Action Discrete : DiscreteIntegrator  SampleTime=SIM.IntegratorSamplingTime  ICPrevOutput=DiscIntNeverNeededParam  ICPrevScaledInput=DiscIntNeverNeededParam
  Sum : Sum  Inputs=|+-
  Sum1 : Sum  Inputs=++|
  Sum2 : Sum  Inputs=|++
  delta_r : Outport
  wires:
  beta_cmd/1 -> Sum/1
  delta_r_trim/1 -> Sum2/2
  Sum1/1 -> Sum2/1  "Ddelta_r"
  Sum/1 -> Gain1/1, Gain/1
  Sum2/1 -> [u_unsat], Rudder Saturation/1
  Gain1/1 -> Sum1/2
  Rudder Saturation/1 -> [u_sat], delta_r/1  "delta_r_sat"
  beta_hat/1 -> Sum/2
  Sideslip I Action Discrete/1 -> Sum1/1
  Gain/1 -> MATLAB Function/3(Ki_e)
  MATLAB Function/1(I) -> Sideslip I Action Discrete/1
  [u_unsat] -> MATLAB Function/1(u_unsat)
  [u_sat] -> MATLAB Function/2(u_sat)

== system Test_Estimation_Effects/Autopilot/Longitudinal Autopilot/Airspeed Hold Control using Pitch Outer Loop ==
  Va_cmd : Inport
  Va_hat : Inport  Port=2
  theta_trim : Inport  Port=3
  Reset_I : Inport  Port=4
  Airspeed Hold using Pitch I Action Discrete : DiscreteIntegrator  ExternalReset=rising  SampleTime=SIM.IntegratorSamplingTime  ICPrevOutput=DiscIntNeverNeededParam  ICPrevScaledInput=DiscIntNeverNeededParam
  Gain1 : Gain  Gain=AP.Airspeed.Pitch.Kp
  Gain2 : Gain  Gain=AP.Airspeed.Pitch.Ki
  MATLAB Function : MATLAB Function  TreatAsAtomicUnit=on
  Pitch CMD Saturation : Saturate  UpperLimit=DES.Airspeed.Pitch.max  LowerLimit=-DES.Airspeed.Pitch.max
  Sum : Sum  Inputs=|+-
  Sum1 : Sum  Inputs=++|
  Sum2 : Sum  Inputs=|++
  pitch_cmd : Outport
  wires:
  Va_cmd/1 -> Sum/1
  Pitch CMD Saturation/1 -> pitch_cmd/1, [u_sat]  "pitch_cmd"
  Sum/1 -> Gain1/1, Gain2/1
  [u_unsat] -> MATLAB Function/1(u_unsat)
  [u_sat] -> MATLAB Function/2(u_sat)
  Gain1/1 -> Sum1/2
  Gain2/1 -> MATLAB Function/3(Ki_e)
  Airspeed Hold using Pitch I Action Discrete/1 -> Sum1/1
  Va_hat/1 -> Sum/2
  theta_trim/1 -> Sum2/2
  Sum1/1 -> Sum2/1  "Dtheta"
  Sum2/1 -> [u_unsat], Pitch CMD Saturation/1
  MATLAB Function/1(I) -> Airspeed Hold using Pitch I Action Discrete/1
  Reset_I/1 -> Airspeed Hold using Pitch I Action Discrete/2

== system Test_Estimation_Effects/Autopilot/Longitudinal Autopilot/Airspeed Hold Control using Throttle  ==
  Va_cmd : Inport
  Va_hat : Inport  Port=2
  delta_t_trim : Inport  Port=3
  Reset_I : Inport  Port=4
  Airspeed Hold using Throttle I Action Discrete : DiscreteIntegrator  ExternalReset=rising  SampleTime=SIM.IntegratorSamplingTime  ICPrevOutput=DiscIntNeverNeededParam  ICPrevScaledInput=DiscIntNeverNeededParam
  Gain1 : Gain  Gain=AP.Airspeed.Throttle.Kp
  Gain2 : Gain  Gain=AP.Airspeed.Throttle.Ki
  MATLAB Function : MATLAB Function  TreatAsAtomicUnit=on
  Sum : Sum  Inputs=|+-
  Sum1 : Sum  Inputs=++|
  Sum2 : Sum  Inputs=|++
  Throttle Saturation : Saturate  UpperLimit=DES.delta_t_max  LowerLimit=0
  delta_t : Outport
  wires:
  Va_hat/1 -> Sum/2
  Airspeed Hold using Throttle I Action Discrete/1 -> Sum1/1
  Gain2/1 -> MATLAB Function/3(Ki_e)
  Gain1/1 -> Sum1/2
  [u_sat] -> MATLAB Function/2(u_sat)
  MATLAB Function/1(I) -> Airspeed Hold using Throttle I Action Discrete/1
  [u_unsat] -> MATLAB Function/1(u_unsat)
  Sum/1 -> Gain2/1, Gain1/1
  Throttle Saturation/1 -> delta_t/1, [u_sat]
  Va_cmd/1 -> Sum/1
  Reset_I/1 -> Airspeed Hold using Throttle I Action Discrete/2
  Sum1/1 -> Sum2/1  "Ddelta_t"
  delta_t_trim/1 -> Sum2/2
  Sum2/1 -> [u_unsat], Throttle Saturation/1

== system Test_Estimation_Effects/Autopilot/Longitudinal Autopilot/Altitude Hold Control Outer Loop ==
  altitude_cmd : Inport
  h_hat : Inport  Port=2
  Reset_I : Inport  Port=3
  theta_trim : Inport  Port=4
  Altitude Hold I Action Discrete : DiscreteIntegrator  ExternalReset=rising  SampleTime=SIM.IntegratorSamplingTime  ICPrevOutput=DiscIntNeverNeededParam  ICPrevScaledInput=DiscIntNeverNeededParam
  Gain1 : Gain  Gain=AP.Altitude.Kp
  Gain2 : Gain  Gain=AP.Altitude.Ki
  MATLAB Function : MATLAB Function  TreatAsAtomicUnit=on
  Pitch CMD Saturation : Saturate  UpperLimit=DES.Altitude.Pitch.max + TRIM.x(8)  LowerLimit=-DES.Altitude.Pitch.max + TRIM.x(8)
  Sum : Sum  Inputs=|+-
  Sum1 : Sum  Inputs=++|
  Sum2 : Sum  Inputs=|++
  pitch_cmd : Outport
  wires:
  Sum/1 -> Gain2/1, Gain1/1
  Sum2/1 -> [u_unsat], Pitch CMD Saturation/1
  Gain2/1 -> MATLAB Function/3(Ki_e)
  Gain1/1 -> Sum1/2
  [u_sat] -> MATLAB Function/2(u_sat)
  Pitch CMD Saturation/1 -> [u_sat], pitch_cmd/1
  [u_unsat] -> MATLAB Function/1(u_unsat)
  altitude_cmd/1 -> Sum/1
  h_hat/1 -> Sum/2
  MATLAB Function/1(I) -> Altitude Hold I Action Discrete/1
  Altitude Hold I Action Discrete/1 -> Sum1/1
  Reset_I/1 -> Altitude Hold I Action Discrete/2
  Sum1/1 -> Sum2/1
  theta_trim/1 -> Sum2/2

== system Test_Estimation_Effects/Autopilot/Longitudinal Autopilot/Pitch Hold Control Loop ==
  pitch_cmd : Inport
  theta_hat : Inport  Port=2
  q_hat : Inport  Port=3
  delta_e_trim : Inport  Port=4
  Elevator Saturation : Saturate  UpperLimit=DES.delta_e_max
  Gain : Gain  Gain=AP.Pitch.Kp
  Gain1 : Gain  Gain=AP.Pitch.Kd
  Sum : Sum  Inputs=|+-
  Sum1 : Sum  Inputs=|+-
  Sum2 : Sum  Inputs=++|
  delta_e : Outport
  wires:
  Gain/1 -> Sum1/1
  Sum/1 -> Gain/1
  Sum2/1 -> Elevator Saturation/1  "delta_e_unsat"
  theta_hat/1 -> Sum/2
  Gain1/1 -> Sum1/2
  Sum1/1 -> Sum2/2  "Ddelta_e"
  delta_e_trim/1 -> Sum2/1
  q_hat/1 -> Gain1/1
  Elevator Saturation/1 -> delta_e/1  "delta_e"
  pitch_cmd/1 -> Sum/1

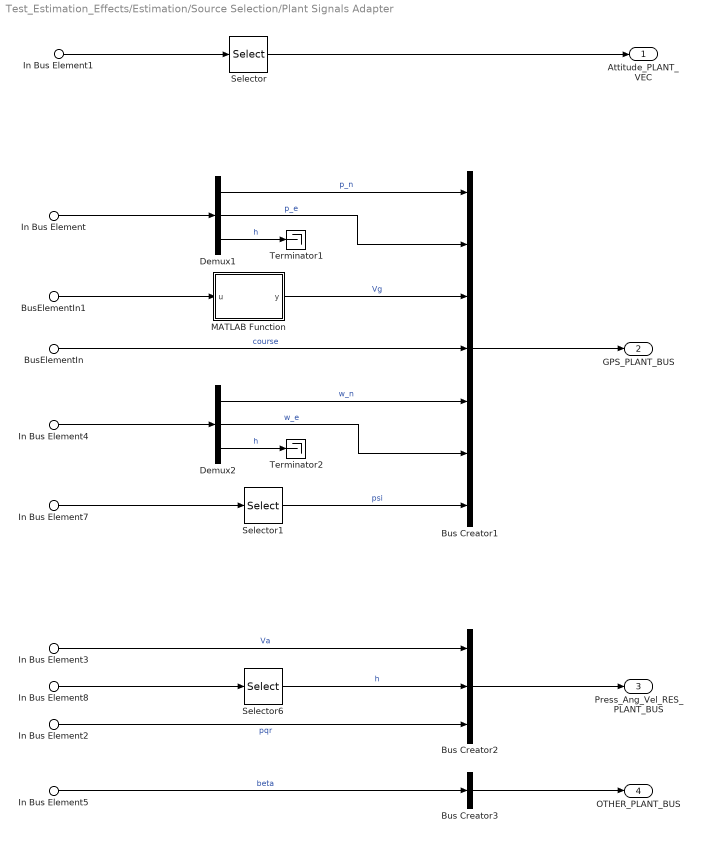
== system Test_Estimation_Effects/Estimation/Source Selection/Plant Signals Adapter ==
  In Bus Element : Inport  PortName=allStates  Element=toSensors.p_neh_inI_3x1
  In Bus Element8 : Inport  PortName=allStates  Element=toSensors.p_neh_inI_3x1
  In Bus Element1 : Inport  PortName=allStates  Element=toSensors.eta_I2B_rad_3x1
  In Bus Element7 : Inport  PortName=allStates  Element=toSensors.eta_I2B_rad_3x1
  In Bus Element2 : Inport  PortName=allStates  Element=toSensors.omega_inB_rad_s_3x1
  In Bus Element4 : Inport  PortName=allStates  Element=toSensors.wind_steady_inI_m_s_3x1
  In Bus Element3 : Inport  PortName=allStates  Element=toSensors.Va
  BusElementIn1 : Inport  PortName=allStates  Element=vg_inB_m_s_3x1
  In Bus Element5 : Inport  PortName=allStates  Element=beta
  BusElementIn : Inport  PortName=allStates  Element=course
  Bus Creator1 : BusCreator  Inputs=7
  Bus Creator2 : BusCreator  Inputs=3
  Bus Creator3 : BusCreator  Inputs=1
  Demux1 : Demux  Outputs=3
  Demux2 : Demux  Outputs=3
  MATLAB Function : MATLAB Function  TreatAsAtomicUnit=on
  Selector : Selector  InputPortWidth=3  IndexOptions=Index vector (dialog)  Indices=[1 2]  OutputSizes=1
  Selector1 : Selector  InputPortWidth=3  IndexOptions=Index vector (dialog)  Indices=[3]  OutputSizes=1
  Selector6 : Selector  InputPortWidth=3  IndexOptions=Index vector (dialog)  Indices=[3]  OutputSizes=1
  Terminator1 : Terminator
  Terminator2 : Terminator
  Attitude_PLANT_VEC : Outport
  GPS_PLANT_BUS : Outport  Port=2
  Press_Ang_Vel_RES_PLANT_BUS : Outport  Port=3
  OTHER_PLANT_BUS : Outport  Port=4
  wires:
  In Bus Element2/1 -> Bus Creator2/3  "pqr"
  In Bus Element4/1 -> Demux2/1
  In Bus Element/1 -> Demux1/1
  Demux1/1 -> Bus Creator1/1  "p_n"
  Demux1/2 -> Bus Creator1/2  "p_e"
  Demux1/3 -> Terminator1/1  "h"
  BusElementIn1/1 -> MATLAB Function/1(u)
  MATLAB Function/1(y) -> Bus Creator1/3  "Vg"
  BusElementIn/1 -> Bus Creator1/4  "course"
  Bus Creator1/1 -> GPS_PLANT_BUS/1
  Demux2/1 -> Bus Creator1/5  "w_n"
  Demux2/2 -> Bus Creator1/6  "w_e"
  Demux2/3 -> Terminator2/1  "h"
  In Bus Element7/1 -> Selector1/1
  Selector1/1 -> Bus Creator1/7  "psi"
  In Bus Element8/1 -> Selector6/1
  In Bus Element3/1 -> Bus Creator2/1  "Va"
  Selector6/1 -> Bus Creator2/2  "h"
  In Bus Element5/1 -> Bus Creator3/1  "beta"
  Bus Creator2/1 -> Press_Ang_Vel_RES_PLANT_BUS/1
  Bus Creator3/1 -> OTHER_PLANT_BUS/1
  In Bus Element1/1 -> Selector/1
  Selector/1 -> Attitude_PLANT_VEC/1

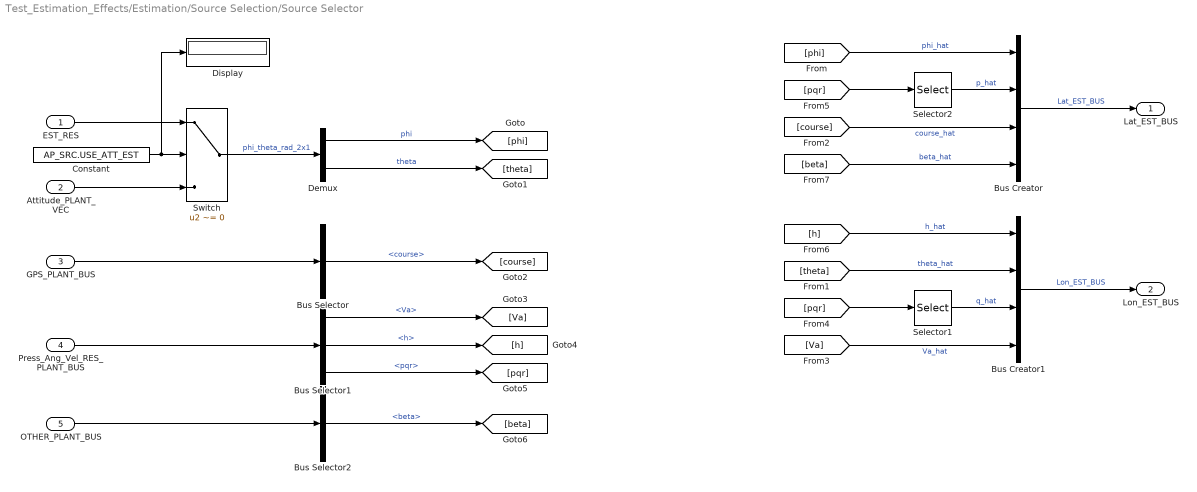
== system Test_Estimation_Effects/Estimation/Source Selection/Source Selector ==
  EST_RES : Inport
  Attitude_PLANT_VEC : Inport  Port=2
  GPS_PLANT_BUS : Inport  Port=3
  Press_Ang_Vel_RES_PLANT_BUS : Inport  Port=4
  OTHER_PLANT_BUS : Inport  Port=5
  Bus Creator : BusCreator  Inputs=4
  Bus Creator1 : BusCreator  Inputs=4
  Bus Selector : BusSelector  OutputSignals=course
  Bus Selector1 : BusSelector  OutputSignals=Va,h,pqr
  Bus Selector2 : BusSelector  OutputSignals=beta
  Constant : Constant  Value=AP_SRC.USE_ATT_EST
  Demux : Demux  Outputs=2
  Display : Display
  Selector1 : Selector  InputPortWidth=3  IndexOptions=Index vector (dialog)  Indices=[2]  OutputSizes=1
  Selector2 : Selector  InputPortWidth=3  IndexOptions=Index vector (dialog)  Indices=[1]  OutputSizes=1
  Switch : Switch  Criteria=u2 ~= 0  SaturateOnIntegerOverflow=off  InputSameDT=off
  Lat_EST_BUS : Outport
  Lon_EST_BUS : Outport  Port=2
  wires:
  [h] -> Bus Creator1/1  "h_hat"
  Selector1/1 -> Bus Creator1/3  "q_hat"
  Bus Creator1/1 -> Lon_EST_BUS/1  "Lon_EST_BUS"
  Selector2/1 -> Bus Creator/2  "p_hat"
  [theta] -> Bus Creator1/2  "theta_hat"
  [Va] -> Bus Creator1/4  "Va_hat"
  [beta] -> Bus Creator/4  "beta_hat"
  Bus Creator/1 -> Lat_EST_BUS/1  "Lat_EST_BUS"
  [phi] -> Bus Creator/1  "phi_hat"
  [course] -> Bus Creator/3  "course_hat"
  Switch/1 -> Demux/1  "phi_theta_rad_2x1"
  Demux/1 -> [phi]  "phi"
  Demux/2 -> [theta]  "theta"
  GPS_PLANT_BUS/1 -> Bus Selector/1
  Bus Selector/1 -> [course]  "<course>"
  Press_Ang_Vel_RES_PLANT_BUS/1 -> Bus Selector1/1
  Bus Selector1/1 -> [Va]  "<Va>"
  Bus Selector1/2 -> [h]  "<h>"
  Bus Selector1/3 -> [pqr]  "<pqr>"
  [pqr] -> Selector1/1
  [pqr] -> Selector2/1
  OTHER_PLANT_BUS/1 -> Bus Selector2/1
  Bus Selector2/1 -> [beta]  "<beta>"
  Attitude_PLANT_VEC/1 -> Switch/3
  EST_RES/1 -> Switch/1
  Constant/1 -> Display/1, Switch/2

== system Test_Estimation_Effects/Plant/Atmospheric Effects/Aerodynamic Effect on Latitude Motion ==
  delta_a : Inport
  delta_r : Inport  Port=2
  beta : Inport  Port=3
  p_r : Inport  Port=4
  Va : Inport  Port=5
  Demux : Demux  Outputs=2
  Demux1 : Demux  Outputs=6
  Demux2 : Demux  Outputs=6
  Demux3 : Demux  Outputs=6
  From : From
  From1 : From
  From2 : From
  Fy : Subsystem
  Goto : Goto
  Mux : Mux  Inputs=3
  Mux1 : Mux  Inputs=6
  Roll Moment (T_p) : Subsystem
  Yaw Moment (T_r) : Subsystem
  Fy_Tp_Tr_inB : Outport
  wires:
  Mux/1 -> Fy_Tp_Tr_inB/1
  p_r/1 -> Demux/1
  Fy/1(Fy_inB_N) -> Mux/1
  Roll Moment (T_p)/1(T_p_inB_Nm) -> Mux/2
  Yaw Moment (T_r)/1(T_r_inB_Nm) -> Mux/3
  Demux1/1 -> Fy/1(delta_a)
  delta_a/1 -> Mux1/1
  delta_r/1 -> Mux1/2
  beta/1 -> Mux1/3
  Demux/1 -> Mux1/4  "p"
  Demux/2 -> Mux1/5  "r"
  Va/1 -> Mux1/6
  Mux1/1 -> Goto/1
  From/1 -> Demux1/1
  Demux1/2 -> Fy/2(delta_r)
  Demux1/3 -> Fy/3(beta)
  Demux1/4 -> Fy/4(p)
  Demux1/5 -> Fy/5(r)
  Demux1/6 -> Fy/6(Va)
  Demux2/4 -> Roll Moment (T_p)/4(p)
  Demux2/5 -> Roll Moment (T_p)/5(r)
  From1/1 -> Demux2/1
  Demux2/2 -> Roll Moment (T_p)/2(delta_r)
  Demux2/1 -> Roll Moment (T_p)/1(delta_a)
  Demux2/6 -> Roll Moment (T_p)/6(Va)
  Demux2/3 -> Roll Moment (T_p)/3(beta)
  Demux3/4 -> Yaw Moment (T_r)/4(p)
  Demux3/5 -> Yaw Moment (T_r)/5(r)
  From2/1 -> Demux3/1
  Demux3/2 -> Yaw Moment (T_r)/2(delta_r)
  Demux3/1 -> Yaw Moment (T_r)/1(delta_a)
  Demux3/6 -> Yaw Moment (T_r)/6(Va)
  Demux3/3 -> Yaw Moment (T_r)/3(beta)

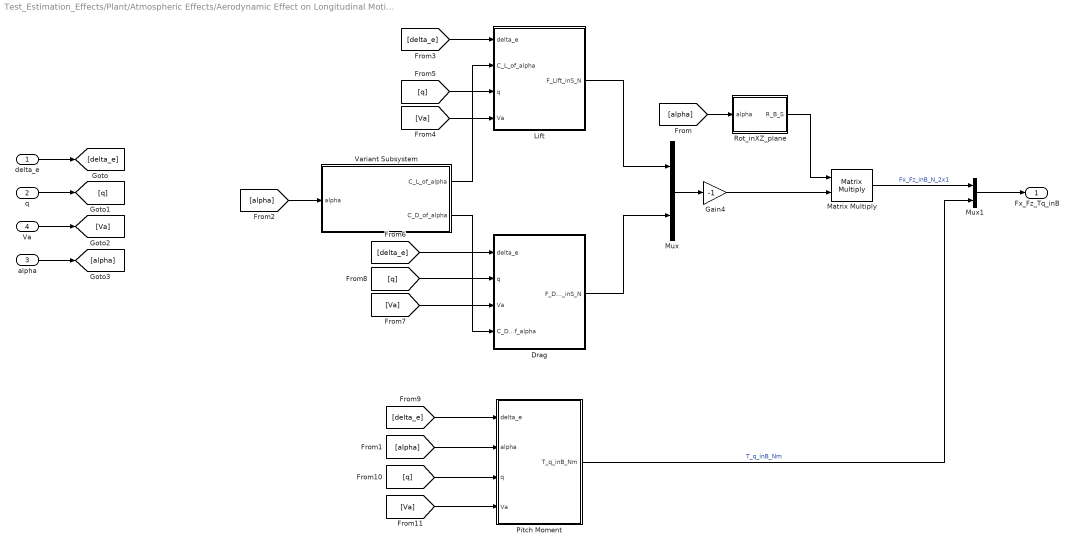
== system Test_Estimation_Effects/Plant/Atmospheric Effects/Aerodynamic Effect on Longitudinal Motion ==
  delta_e : Inport
  q : Inport  Port=2
  alpha : Inport  Port=3
  Va : Inport  Port=4
  Drag : Subsystem
  Gain4 : Gain  Gain=-1
  "Lift " : Subsystem
  Matrix Multiply : Product  Multiplication=Matrix(*)
  Mux : Mux  Inputs=2
  Mux1 : Mux  Inputs=2
  Pitch Moment : Subsystem
  Rot_inXZ_plane : MATLAB Function  TreatAsAtomicUnit=on
  Variant Subsystem : Subsystem  Variant=on
  Fx_Fz_Tq_inB : Outport
  wires:
  alpha/1 -> [alpha]
  [alpha] -> Rot_inXZ_plane/1(alpha)
  Mux/1 -> Gain4/1
  Rot_inXZ_plane/1(R_B_S) -> Matrix Multiply/1
  Gain4/1 -> Matrix Multiply/2
  Matrix Multiply/1 -> Mux1/1  "Fx_Fz_inB_N_2x1"
  Variant Subsystem/1(C_L_of_alpha) -> "Lift "/2(C_L_of_alpha)
  "Lift "/1(F_Lift_inS_N) -> Mux/1
  Variant Subsystem/2(C_D_of_alpha) -> Drag/4(C_D_of_alpha)
  Drag/1(F_Drag_inS_N) -> Mux/2
  Pitch Moment/1(T_q_inB_Nm) -> Mux1/2  "T_q_inB_Nm"
  Mux1/1 -> Fx_Fz_Tq_inB/1
  delta_e/1 -> [delta_e]
  Va/1 -> [Va]
  q/1 -> [q]
  [alpha] -> Variant Subsystem/1(alpha)
  [delta_e] -> "Lift "/1(delta_e)
  [Va] -> "Lift "/4(Va)
  [q] -> "Lift "/3(q)
  [delta_e] -> Drag/1(delta_e)
  [q] -> Drag/2(q)
  [Va] -> Drag/3(Va)
  [delta_e] -> Pitch Moment/1(delta_e)
  [q] -> Pitch Moment/3(q)
  [Va] -> Pitch Moment/4(Va)
  [alpha] -> Pitch Moment/2(alpha)

== system Test_Estimation_Effects/Plant/Subsystem1/Subsystem ==
  eta_I2B_rad_3x1 : Inport
  MATLAB Function : MATLAB Function  TreatAsAtomicUnit=on
  T_3x3 : Outport
  wires:
  eta_I2B_rad_3x1/1 -> MATLAB Function/1(u)
  MATLAB Function/1(y) -> T_3x3/1

== system Test_Estimation_Effects/Plant/Va-Alpha-Beta Extraction/norm2 ==
  Va_inB_m_s_3x1 : Inport
  Sqrt : Sqrt
  Square : Math  Operator=square
  Sum of Elements : Sum  Inputs=+
  Va : Outport
  wires:
  Va_inB_m_s_3x1/1 -> Square/1
  Square/1 -> Sum of Elements/1
  Sum of Elements/1 -> Sqrt/1
  Sqrt/1 -> Va/1

== system Test_Estimation_Effects/Autopilot/Lateral Autopilot/Course Hold Control Loop/Roll Hold Control Loop ==
  phi_cmd : Inport
  delta_a_trim : Inport  Port=2
  phi_hat : Inport  Port=3
  p_hat : Inport  Port=4
  Aileron Saturation : Saturate  UpperLimit=DES.delta_a_max  LowerLimit=-DES.delta_a_max
  Gain1 : Gain  Gain=AP.Roll.Kp
  Gain2 : Gain  Gain=-AP.Roll.Kd
  Gain3 : Gain  Gain=AP.Roll.Ki
  MATLAB Function : MATLAB Function  TreatAsAtomicUnit=on
  Roll I Action Discrete : DiscreteIntegrator  SampleTime=SIM.IntegratorSamplingTime  ICPrevOutput=DiscIntNeverNeededParam  ICPrevScaledInput=DiscIntNeverNeededParam
  Sum : Sum  Inputs=|++
  Sum1 : Sum  Inputs=|+-
  Sum2 : Sum  Inputs=+++
  delta_a_sat : Outport
  wires:
  phi_cmd/1 -> Sum1/1
  Sum1/1 -> Gain1/1, Gain3/1
  Sum2/1 -> Sum/1  "Ddelta_a_unsat"
  phi_hat/1 -> Sum1/2
  p_hat/1 -> Gain2/1
  [u_unsat] -> MATLAB Function/1(u_unsat)
  [u_sat] -> MATLAB Function/2(u_sat)
  MATLAB Function/1(I) -> Roll I Action Discrete/1
  Roll I Action Discrete/1 -> Sum2/1
  Gain1/1 -> Sum2/2
  Gain2/1 -> Sum2/3
  delta_a_trim/1 -> Sum/2
  Sum/1 -> Aileron Saturation/1, [u_unsat]
  Aileron Saturation/1 -> delta_a_sat/1, [u_sat]
  Gain3/1 -> MATLAB Function/3(Ki_e)

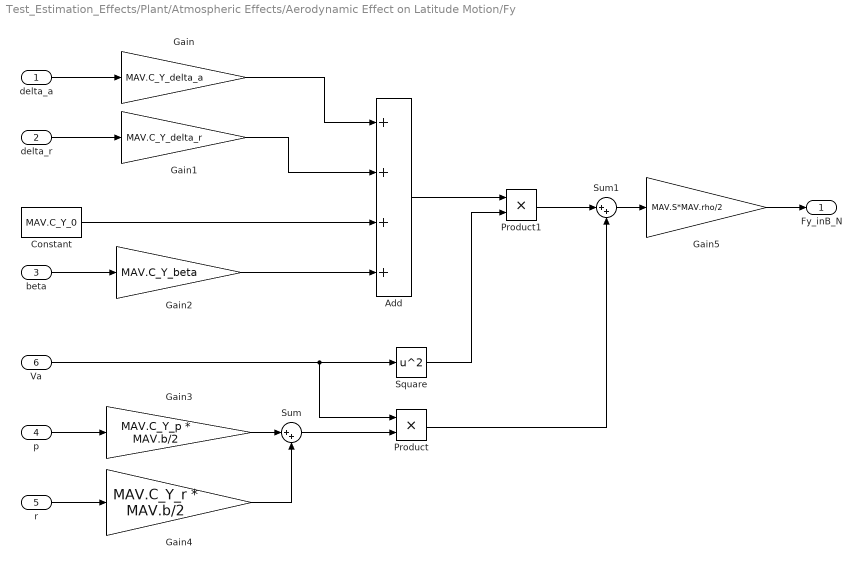
== system Test_Estimation_Effects/Plant/Atmospheric Effects/Aerodynamic Effect on Latitude Motion/Fy ==
  delta_a : Inport
  delta_r : Inport  Port=2
  beta : Inport  Port=3
  p : Inport  Port=4
  r : Inport  Port=5
  Va : Inport  Port=6
  Add : Sum  Inputs=++++
  Constant : Constant  Value=MAV.C_Y_0
  Gain : Gain  Gain=MAV.C_Y_delta_a
  Gain1 : Gain  Gain=MAV.C_Y_delta_r
  Gain2 : Gain  Gain=MAV.C_Y_beta
  Gain3 : Gain  Gain=MAV.C_Y_p * MAV.b/2
  Gain4 : Gain  Gain=MAV.C_Y_r * MAV.b/2
  Gain5 : Gain  Gain=MAV.S*MAV.rho/2
  Product : Product
  Product1 : Product
  Square : Math  Operator=square
  Sum : Sum  Inputs=|++
  Sum1 : Sum  Inputs=|++
  Fy_inB_N : Outport
  wires:
  delta_a/1 -> Gain/1
  delta_r/1 -> Gain1/1
  Constant/1 -> Add/3
  beta/1 -> Gain2/1
  Gain2/1 -> Add/4
  p/1 -> Gain3/1
  r/1 -> Gain4/1
  Gain3/1 -> Sum/1
  Gain4/1 -> Sum/2
  Gain/1 -> Add/1
  Gain1/1 -> Add/2
  Sum/1 -> Product/2
  Va/1 -> Square/1, Product/1
  Add/1 -> Product1/1
  Square/1 -> Product1/2
  Product1/1 -> Sum1/1
  Product/1 -> Sum1/2
  Sum1/1 -> Gain5/1
  Gain5/1 -> Fy_inB_N/1

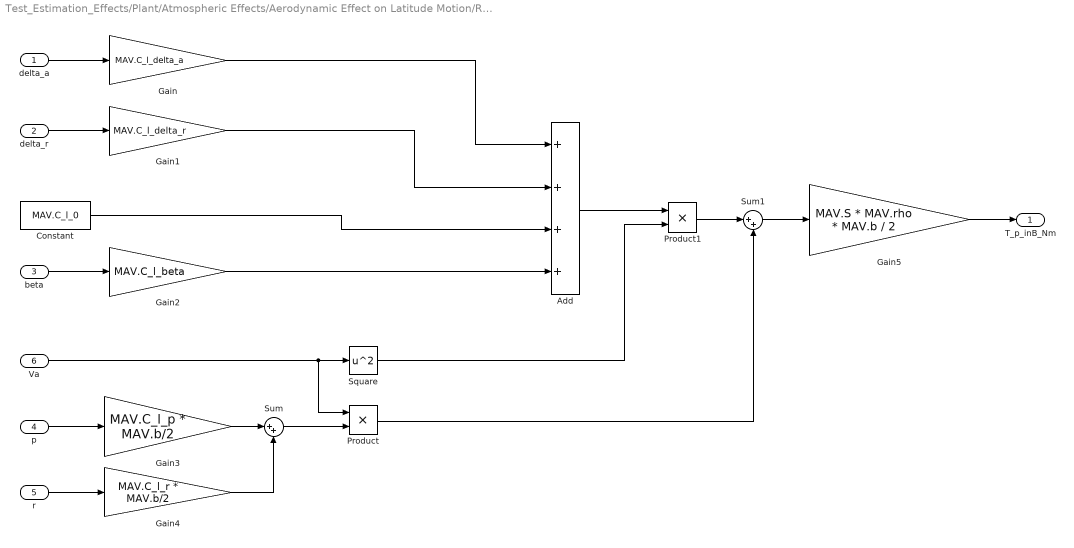
== system Test_Estimation_Effects/Plant/Atmospheric Effects/Aerodynamic Effect on Latitude Motion/Roll Moment (T_p) ==
  delta_a : Inport
  delta_r : Inport  Port=2
  beta : Inport  Port=3
  p : Inport  Port=4
  r : Inport  Port=5
  Va : Inport  Port=6
  Add : Sum  Inputs=++++
  Constant : Constant  Value=MAV.C_l_0
  Gain : Gain  Gain=MAV.C_l_delta_a
  Gain1 : Gain  Gain=MAV.C_l_delta_r
  Gain2 : Gain  Gain=MAV.C_l_beta
  Gain3 : Gain  Gain=MAV.C_l_p * MAV.b/2
  Gain4 : Gain  Gain=MAV.C_l_r * MAV.b/2
  Gain5 : Gain  Gain=MAV.S * MAV.rho * MAV.b / 2
  Product : Product
  Product1 : Product
  Square : Math  Operator=square
  Sum : Sum  Inputs=|++
  Sum1 : Sum  Inputs=|++
  T_p_inB_Nm : Outport
  wires:
  Gain1/1 -> Add/2
  Gain/1 -> Add/1
  Va/1 -> Square/1, Product/1
  Sum/1 -> Product/2
  Gain4/1 -> Sum/2
  Gain3/1 -> Sum/1
  r/1 -> Gain4/1
  p/1 -> Gain3/1
  Gain2/1 -> Add/4
  beta/1 -> Gain2/1
  Constant/1 -> Add/3
  delta_r/1 -> Gain1/1
  delta_a/1 -> Gain/1
  Add/1 -> Product1/1
  Square/1 -> Product1/2
  Product1/1 -> Sum1/1
  Product/1 -> Sum1/2
  Sum1/1 -> Gain5/1
  Gain5/1 -> T_p_inB_Nm/1

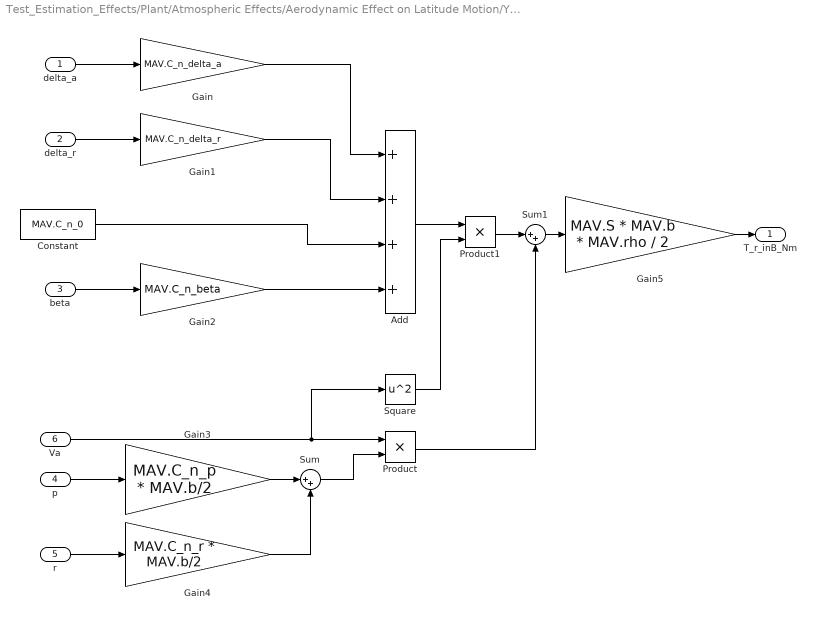
== system Test_Estimation_Effects/Plant/Atmospheric Effects/Aerodynamic Effect on Latitude Motion/Yaw Moment (T_r) ==
  delta_a : Inport
  delta_r : Inport  Port=2
  beta : Inport  Port=3
  p : Inport  Port=4
  r : Inport  Port=5
  Va : Inport  Port=6
  Add : Sum  Inputs=++++
  Constant : Constant  Value=MAV.C_n_0
  Gain : Gain  Gain=MAV.C_n_delta_a
  Gain1 : Gain  Gain=MAV.C_n_delta_r
  Gain2 : Gain  Gain=MAV.C_n_beta
  Gain3 : Gain  Gain=MAV.C_n_p * MAV.b/2
  Gain4 : Gain  Gain=MAV.C_n_r * MAV.b/2
  Gain5 : Gain  Gain=MAV.S * MAV.b * MAV.rho / 2
  Product : Product
  Product1 : Product
  Square : Math  Operator=square
  Sum : Sum  Inputs=|++
  Sum1 : Sum  Inputs=|++
  T_r_inB_Nm : Outport
  wires:
  Gain2/1 -> Add/4
  Constant/1 -> Add/3
  Gain1/1 -> Add/2
  delta_a/1 -> Gain/1
  p/1 -> Gain3/1
  Sum/1 -> Product/2
  Gain/1 -> Add/1
  r/1 -> Gain4/1
  Va/1 -> Square/1, Product/1
  Gain3/1 -> Sum/1
  delta_r/1 -> Gain1/1
  beta/1 -> Gain2/1
  Gain4/1 -> Sum/2
  Add/1 -> Product1/1
  Square/1 -> Product1/2
  Product1/1 -> Sum1/1
  Product/1 -> Sum1/2
  Sum1/1 -> Gain5/1
  Gain5/1 -> T_r_inB_Nm/1

== system Test_Estimation_Effects/Plant/Atmospheric Effects/Aerodynamic Effect on Longitudinal Motion/Drag ==
  delta_e : Inport
  q : Inport  Port=2
  Va : Inport  Port=3
  C_D_of_alpha : Inport  Port=4
  Gain : Gain  Gain=MAV.S * MAV.rho / 2
  Gain2 : Gain  Gain=MAV.C_D_delta_e
  Gain3 : Gain  Gain=MAV.C_D_q * MAV.c / 2
  Product : Product
  Product1 : Product
  Square : Math  Operator=square
  Sum : Sum  Inputs=|++
  Sum1 : Sum  Inputs=|++
  F_Drag_inS_N : Outport
  wires:
  Gain2/1 -> Sum/2
  delta_e/1 -> Gain2/1
  C_D_of_alpha/1 -> Sum/1
  q/1 -> Gain3/1
  Va/1 -> Square/1, Product/1
  Gain3/1 -> Product/2
  Sum/1 -> Product1/1
  Square/1 -> Product1/2
  Product1/1 -> Sum1/1
  Product/1 -> Sum1/2
  Sum1/1 -> Gain/1
  Gain/1 -> F_Drag_inS_N/1

== system Test_Estimation_Effects/Plant/Atmospheric Effects/Aerodynamic Effect on Longitudinal Motion/Lift  ==
  delta_e : Inport
  C_L_of_alpha : Inport  Port=2
  q : Inport  Port=3
  Va : Inport  Port=4
  Gain : Gain  Gain=MAV.C_L_delta_e
  Gain1 : Gain  Gain=MAV.C_L_q * MAV.c / 2
  Gain2 : Gain  Gain=MAV.S * MAV.rho / 2
  Product : Product
  Product1 : Product
  Square : Math  Operator=square
  Sum : Sum  Inputs=|++
  Sum1 : Sum  Inputs=|++
  F_Lift_inS_N : Outport
  wires:
  Gain/1 -> Sum/1
  C_L_of_alpha/1 -> Sum/2
  delta_e/1 -> Gain/1
  q/1 -> Gain1/1
  Gain1/1 -> Product/2
  Va/1 -> Product/1, Square/1
  Sum/1 -> Product1/1
  Square/1 -> Product1/2
  Product1/1 -> Sum1/1
  Product/1 -> Sum1/2
  Sum1/1 -> Gain2/1
  Gain2/1 -> F_Lift_inS_N/1
